simulink model "DualActiveBridgeConverter"  (R2026a)
settings: Solver=ode23t  StopTime=0.010  MaxStep=1e-5  AbsTol=1e-3
PreLoadFcn:
  | DABDefaultInputParameters;
model workspace (MAT data in the model file):
  ConverterKey : string (value not decoded)
undefined symbols (not defined in the file): DABController, DABDesign
libraries: ee_lib x45, nesl_utility x38, fl_lib x19, ConverterLibrary x1, simulink_extras x1
(part 2 of 5)

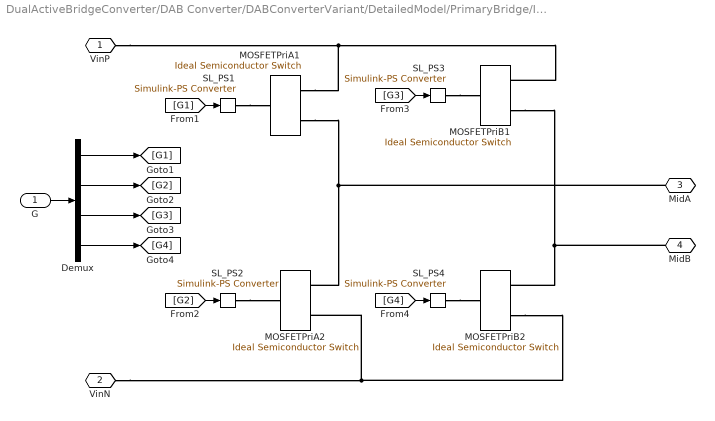
== system DualActiveBridgeConverter/DAB Converter/DABConverterVariant/DetailedModel/PrimaryBridge/IdealSwitch ==
  G : Inport
  Demux : Demux
  MOSFETPriA1 : ee_lib/Semiconductors & Converters/Ideal Semiconductor Switch  port_option=ee.enum.controlport.ps  Ron=RdsOnPri_SI Ohm  Goff=GdsOffPri_SI 1/Ohm  Vth=VthPri_SI V  diode_param=ee.enum.semiconductors.protectionDiode.nodynamics  diode_Vf=VfPri_SI V  diode_Ron=RdPri_SI Ohm  diode_Goff=GdPri_SI 1/Ohm  diode_C=50e-9 F  diode_iRM=-235 A  diode_iF=300 A  diode_idot=-50 A/us  diode_trr_param=ee.enum.converters.diodetrr.trr_factor  diode_trr_factor=3  diode_trr=15 us  diode_Qrr=1500 s*uA
  MOSFETPriA2 : ee_lib/Semiconductors & Converters/Ideal Semiconductor Switch  port_option=ee.enum.controlport.ps  Ron=RdsOnPri_SI Ohm  Goff=GdsOffPri_SI 1/Ohm  Vth=VthPri_SI V  diode_param=ee.enum.semiconductors.protectionDiode.nodynamics  diode_Vf=VfPri_SI V  diode_Ron=RdPri_SI Ohm  diode_Goff=GdPri_SI 1/Ohm  diode_C=50e-9 F  diode_iRM=-235 A  diode_iF=300 A  diode_idot=-50 A/us  diode_trr_param=ee.enum.converters.diodetrr.trr_factor  diode_trr_factor=3  diode_trr=15 us  diode_Qrr=1500 s*uA
  MOSFETPriB1 : ee_lib/Semiconductors & Converters/Ideal Semiconductor Switch  port_option=ee.enum.controlport.ps  Ron=RdsOnPri_SI Ohm  Goff=GdsOffPri_SI 1/Ohm  Vth=VthPri_SI V  diode_param=ee.enum.semiconductors.protectionDiode.nodynamics  diode_Vf=VfPri_SI V  diode_Ron=RdPri_SI Ohm  diode_Goff=GdPri_SI 1/Ohm  diode_C=50e-9 F  diode_iRM=-235 A  diode_iF=300 A  diode_idot=-50 A/us  diode_trr_param=ee.enum.converters.diodetrr.trr_factor  diode_trr_factor=3  diode_trr=15 us  diode_Qrr=1500 s*uA
  MOSFETPriB2 : ee_lib/Semiconductors & Converters/Ideal Semiconductor Switch  port_option=ee.enum.controlport.ps  Ron=RdsOnPri_SI Ohm  Goff=GdsOffPri_SI 1/Ohm  Vth=VthPri_SI V  diode_param=ee.enum.semiconductors.protectionDiode.nodynamics  diode_Vf=VfPri_SI V  diode_Ron=RdPri_SI Ohm  diode_Goff=GdPri_SI 1/Ohm  diode_C=50e-9 F  diode_iRM=-235 A  diode_iF=300 A  diode_idot=-50 A/us  diode_trr_param=ee.enum.converters.diodetrr.trr_factor  diode_trr_factor=3  diode_trr=15 us  diode_Qrr=1500 s*uA
  SL_PS{1..4} (4 alike) : nesl_utility/Simulink-PS Converter  PhysicalDomain=network_engine_domain  SubClassName=ps_input  LeftPortType=input  RightPortType=output  PseudoPeriodic=off  Frequencies=[]  NoiseDistribution=none  NoiseParameters=[]  Unit=1  AffineConversion=off  FilteringAndDerivatives=provide  SimscapeFilterOrder=1  InputFilterTimeConstant=0.001  UdotUserProvided=0
  VinP : PMIOPort  Side=Left
  VinN : PMIOPort  Port=2  Side=Left
  MidA : PMIOPort  Port=3  Side=Right
  MidB : PMIOPort  Port=4  Side=Right
  wires:
  G/1 -> Demux/1
  Demux/1 -> [G1]
  Demux/2 -> [G2]
  Demux/3 -> [G3]
  Demux/4 -> [G4]
  [G1] -> SL_PS1/1
  [G2] -> SL_PS2/1
  [G3] -> SL_PS3/1
  [G4] -> SL_PS4/1
  connections:
  SL_PS4/RConn1 -- MOSFETPriB2/LConn1
  SL_PS3/RConn1 -- MOSFETPriB1/LConn1
  SL_PS2/RConn1 -- MOSFETPriA2/LConn1
  SL_PS1/RConn1 -- MOSFETPriA1/LConn1
  VinP/RConn1 -- MOSFETPriA1/RConn1 -- MOSFETPriB1/RConn1
  MOSFETPriB1/RConn2 -- MidB/RConn1 -- MOSFETPriB2/RConn1
  MOSFETPriA1/RConn2 -- MOSFETPriA2/RConn1 -- MidA/RConn1
  VinN/RConn1 -- MOSFETPriB2/RConn2 -- MOSFETPriA2/RConn2
